simulink model "hover"  (R2025a)
settings: Solver=ode1  StopTime=160  FixedStep=Ts
InitFcn:
  | StartParameters
undefined symbols (not defined in the file or in its folder): enableOriginalWind, K_v4Hover, nL_eq, nR_eq, q0, qp0, tauL_eq, tauR_eq, Ts
settings Model: Creator=pedro  LastModifiedBy=pedro55562
settings SolverCC: AlgebraicLoopSolver=TrustRegion
settings DataIOCC: LimitDataPoints=on  SaveFormat=Array  SignalLoggingSaveFormat=ModelDataLogs  ReturnWorkspaceOutputs=off
settings OptimizationCC: BlockReduction=off  BooleanDataType=off  LifeSpan=inf
settings DebuggingCC: SaveWithParameterizedLinksMsg=none  SignalResolutionControl=TryResolveAllWithWarning  MultiTaskDSMMsg=warning  MultiTaskCondExecSysMsg=none  UnconnectedInputMsg=warning  UnconnectedOutputMsg=warning  UnconnectedLineMsg=warning  StateNameClashWarn=warning  SFUnexpectedBacktrackingDiag=warning  SFNoUnconditionalDefaultTransitionDiag=warning  SFExecutionAtInitializationDiag=none  ArithmeticOperatorsInVariantConditions=warning
settings HardwareCC: ProdBitPerPointer=32.0  ProdBitPerSizeT=32.0  ProdBitPerPtrDiffT=32.0  ProdLargestAtomicFloat=None  ProdIntDivRoundTo=Undefined  ProdEndianess=Unspecified  ProdWordSize=32.0  ProdHWDeviceType=32-bit Generic
settings SFSimCC: SimGPUStackLimitPerThread=51200  SimGPUMallocThreshold=200
settings RTWCC: GPUStackLimitPerThread=51200  GPUMallocThreshold=200

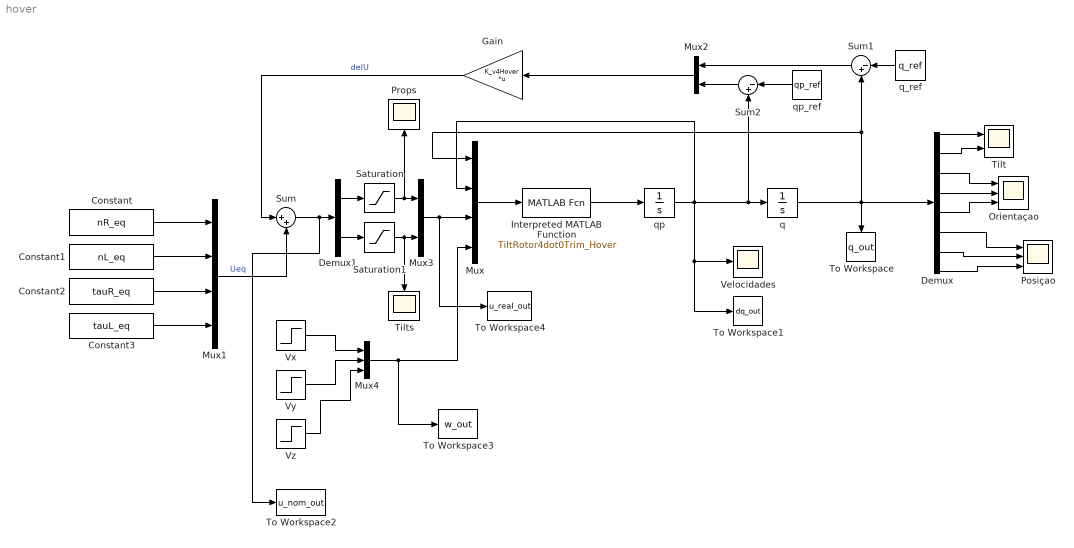
== system hover ==
  Constant : Constant  Value=nR_eq
  Constant1 : Constant  Value=nL_eq
  Constant2 : Constant  Value=tauR_eq
  Constant3 : Constant  Value=tauL_eq
  Demux : Demux  Outputs=8
  Demux1 : Demux  Outputs=2
  Gain : Gain  Gain=K_v4Hover  Multiplication=Matrix(K*u)
  Interpreted MATLAB Function : MATLABFcn  MATLABFcn=TiltRotor4dot0Trim_Hover
  Mux : Mux
  Mux1 : Mux
  Mux2 : Mux  Inputs=2
  Mux3 : Mux  Inputs=2
  Mux4 : Mux  Inputs=3
  Orientaçao : Scope  NumInputPorts=3
      settings: ActiveDisplayYMinimum=-0.358  ActiveDisplayYMaximum=0.50584
  Posiçao : Scope  NumInputPorts=3
      settings: ActiveDisplayYMinimum=-1.20947  ActiveDisplayYMaximum=1.7096  DataLoggingVariableName=ScopeData2
  Props : Scope
      settings: ActiveDisplayYMinimum=42.2448  ActiveDisplayYMaximum=58.93016  DataLoggingVariableName=ScopeData4
  Saturation : Saturate  UpperLimit=100  LowerLimit=0
  Saturation1 : Saturate  UpperLimit=10  LowerLimit=-10
  Sum : Sum  Inputs=|++
  Sum1 : Sum  Inputs=|-+
  Sum2 : Sum  Inputs=|-+
  Tilt : Scope  NumInputPorts=2
      settings: ActiveDisplayYMinimum=-0.35418  ActiveDisplayYMaximum=-0.07091  DataLoggingVariableName=ScopeData3
  Tilts : Scope
      settings: ActiveDisplayYMinimum=-2.71878  ActiveDisplayYMaximum=0.19588  DataLoggingVariableName=ScopeData5
  To Workspace : ToWorkspace  VariableName=q_out  SaveFormat=Structure With Time  SampleTime=Ts
  To Workspace1 : ToWorkspace  VariableName=dq_out  SaveFormat=Structure With Time  SampleTime=Ts
  To Workspace2 : ToWorkspace  VariableName=u_nom_out  SaveFormat=Structure With Time  SampleTime=Ts
  To Workspace3 : ToWorkspace  VariableName=w_out  SaveFormat=Structure With Time  SampleTime=Ts
  To Workspace4 : ToWorkspace  VariableName=u_real_out  SaveFormat=Structure With Time  SampleTime=Ts
  Velocidades : Scope
      settings: ActiveDisplayYMinimum=-30.24551  ActiveDisplayYMaximum=17.03382
  Vx : Step  Time=10  After=5*enableOriginalWind  SampleTime=0
  Vy : Step  Time=60  After=5*enableOriginalWind  SampleTime=0
  Vz : Step  Time=110  After=5*enableOriginalWind  SampleTime=0
  q : Integrator  InitialCondition=q0'
  q_ref : FromWorkspace  VariableName=q_ref  SampleTime=Ts  OutputAfterFinalValue=Holding final value
  "qp " : Integrator  InitialCondition=qp0'
  qp_ref : FromWorkspace  VariableName=qp_ref  SampleTime=Ts  OutputAfterFinalValue=Holding final value
  wires:
  Interpreted MATLAB Function/1 -> "qp "/1
  Mux/1 -> Interpreted MATLAB Function/1
  "qp "/1 -> Mux/2, Sum2/2, q/1, To Workspace1/1, Velocidades/1
  Constant/1 -> Mux1/1
  Constant1/1 -> Mux1/2
  Constant2/1 -> Mux1/3
  Constant3/1 -> Mux1/4
  Mux1/1 -> Sum/2  "Ueq"
  Gain/1 -> Sum/1  "delU"
  Mux2/1 -> Gain/1
  q_ref/1 -> Sum1/1
  Sum1/1 -> Mux2/1
  qp_ref/1 -> Sum2/1
  Sum2/1 -> Mux2/2
  q/1 -> To Workspace/1, Demux/1, Sum1/2, Mux/1
  Mux4/1 -> To Workspace3/1, Mux/4
  Vx/1 -> Mux4/1
  Vy/1 -> Mux4/2
  Vz/1 -> Mux4/3
  Demux/7 -> Posiçao/2
  Demux/1 -> Tilt/1
  Demux/5 -> Orientaçao/3
  Demux/6 -> Posiçao/1
  Demux/8 -> Posiçao/3
  Demux/3 -> Orientaçao/1
  Demux/4 -> Orientaçao/2
  Demux/2 -> Tilt/2
  Sum/1 -> To Workspace2/1, Demux1/1
  Demux1/1 -> Saturation/1
  Saturation/1 -> Props/1, Mux3/1
  Saturation1/1 -> Tilts/1, Mux3/2
  Demux1/2 -> Saturation1/1
  Mux3/1 -> To Workspace4/1, Mux/3
